simulink model "s_b4a4x32kf_26"  (R2018a)
settings: Solver=VariableStepDiscrete  StartTime=0.0  StopTime=10000  RelTol=1e-3
undefined symbols (not defined in the file): fft_stages, n_bits_ants, n_bits_xengs
libraries: xbsIndex_r4 x21247, casper_library_misc x37, casper_library_scopes x13, casper_library_delays x8, xbsReplacements_r4 x6, xps_library x4
(part 44 of 268)

== system s_b4a4x32kf_26/sys2/xeng_tvg ==
  sync : Inport
  data_in : Inport  Port=2
  valid_in : Inport  Port=3
  mcnti : Inport  Port=4
  Concat1 : xbsIndex_r4/Concat  num_inputs=4  dbl_ovrd=off  block_type=concat
      settings: SourceProductName=The database /home/jmanley/.matlab/R2018a/slblocks_master.db is locked, or a table in the database is locked. (database is locked)  block_version=10.1.3
  Constant1 : xbsIndex_r4/Constant  const=0.75  gui_display_data_type=Fixed-point  arith_type=Signed (2's comp)  n_bits=n_bits  bin_pt=n_bits-1  preci_type=Single  exp_width=8  frac_width=24  explicit_period=on  period=1  equ=P=C  opselect=C  inp2=PCIN>>17  opr=+  inp1=P  carry=CIN  dbl_ovrd=off  block_type=constant
      settings: SourceProductName=The database /home/jmanley/.matlab/R2018a/slblocks_master.db is locked, or a table in the database is locked. (database is locked)
  Constant13 : xbsIndex_r4/Constant  const=1  gui_display_data_type=Fixed-point  arith_type=Boolean  n_bits=1  bin_pt=0  preci_type=Single  exp_width=8  frac_width=24  explicit_period=on  period=1  equ=P=C  opselect=C  inp2=PCIN>>17  opr=+  inp1=P  carry=CIN  dbl_ovrd=off  block_type=constant
      settings: SourceProductName=The database /home/jmanley/.matlab/R2018a/slblocks_master.db is locked, or a table in the database is locked. (database is locked)
  Constant2 : xbsIndex_r4/Constant  const=0.125  gui_display_data_type=Fixed-point  arith_type=Signed (2's comp)  n_bits=n_bits  bin_pt=n_bits-1  preci_type=Single  exp_width=8  frac_width=24  explicit_period=on  period=1  equ=P=C  opselect=C  inp2=PCIN>>17  opr=+  inp1=P  carry=CIN  dbl_ovrd=off  block_type=constant
      settings: SourceProductName=The database /home/jmanley/.matlab/R2018a/slblocks_master.db is locked, or a table in the database is locked. (database is locked)
  Constant4 : xbsIndex_r4/Constant  const=-0.25  gui_display_data_type=Fixed-point  arith_type=Signed (2's comp)  n_bits=n_bits  bin_pt=n_bits-1  preci_type=Single  exp_width=8  frac_width=24  explicit_period=on  period=1  equ=P=C  opselect=C  inp2=PCIN>>17  opr=+  inp1=P  carry=CIN  dbl_ovrd=off  block_type=constant
      settings: SourceProductName=The database /home/jmanley/.matlab/R2018a/slblocks_master.db is locked, or a table in the database is locked. (database is locked)
  Constant7 : xbsIndex_r4/Constant  const=0.25  gui_display_data_type=Fixed-point  arith_type=Signed (2's comp)  n_bits=n_bits  bin_pt=n_bits-1  preci_type=Single  exp_width=8  frac_width=24  explicit_period=on  period=1  equ=P=C  opselect=C  inp2=PCIN>>17  opr=+  inp1=P  carry=CIN  dbl_ovrd=off  block_type=constant
      settings: SourceProductName=The database /home/jmanley/.matlab/R2018a/slblocks_master.db is locked, or a table in the database is locked. (database is locked)
  Counter : xbsIndex_r4/Counter  cnt_type=Free Running  cnt_to=Inf  operation=Up  start_count=0  cnt_by_val=1  arith_type=Unsigned  n_bits=x_int_bits + 1  bin_pt=0  load_pin=off  rst=on  en=off  explicit_period=off  period=1  use_behavioral_HDL=off  implementation=Fabric  use_rpm=on  dbl_ovrd=off  block_type=counter
      settings: SourceProductName=The database /home/jmanley/.matlab/R2018a/slblocks_master.db is locked, or a table in the database is locked. (database is locked)  xl_area=[0, 0, 0, 0, 0, 0, 0]
  Counter1 : xbsIndex_r4/Counter  cnt_type=Free Running  cnt_to=7  operation=Up  start_count=0  cnt_by_val=1  arith_type=Unsigned  n_bits=n_bits  bin_pt=0  load_pin=off  rst=on  en=on  explicit_period=off  period=1  use_behavioral_HDL=off  implementation=Fabric  use_rpm=on  dbl_ovrd=off  block_type=counter
      settings: SourceProductName=The database /home/jmanley/.matlab/R2018a/slblocks_master.db is locked, or a table in the database is locked. (database is locked)  xl_area=[0, 0, 0, 0, 0, 0, 0]
  Counter2 : xbsIndex_r4/Counter  cnt_type=Free Running  cnt_to=Inf  operation=Up  start_count=0  cnt_by_val=1  arith_type=Unsigned  n_bits=mcnt_period+1  bin_pt=0  load_pin=off  rst=on  en=on  explicit_period=off  period=1  use_behavioral_HDL=off  implementation=Fabric  use_rpm=on  dbl_ovrd=off  block_type=counter
      settings: SourceProductName=The database /home/jmanley/.matlab/R2018a/slblocks_master.db is locked, or a table in the database is locked. (database is locked)  xl_area=[0, 0, 0, 0, 0, 0, 0]
  Counter3 : xbsIndex_r4/Counter  cnt_type=Free Running  cnt_to=0  operation=Down  start_count=2^n_bits-1  cnt_by_val=1  arith_type=Unsigned  n_bits=n_bits  bin_pt=0  load_pin=off  rst=on  en=on  explicit_period=off  period=1  use_behavioral_HDL=off  implementation=Fabric  use_rpm=on  dbl_ovrd=off  block_type=counter
      settings: SourceProductName=The database /home/jmanley/.matlab/R2018a/slblocks_master.db is locked, or a table in the database is locked. (database is locked)  xl_area=[0, 0, 0, 0, 0, 0, 0]
  Counter4 : xbsIndex_r4/Counter  cnt_type=Free Running  cnt_to=Inf  operation=Up  start_count=2^sync_period - 2  cnt_by_val=1  arith_type=Unsigned  n_bits=sync_period+1  bin_pt=0  load_pin=off  rst=off  en=off  explicit_period=off  period=1  use_behavioral_HDL=off  implementation=Fabric  use_rpm=on  dbl_ovrd=off  block_type=counter
      settings: SourceProductName=The database /home/jmanley/.matlab/R2018a/slblocks_master.db is locked, or a table in the database is locked. (database is locked)  xl_area=[0, 0, 0, 0, 0, 0, 0]
  Counter5 : xbsIndex_r4/Counter  cnt_type=Free Running  cnt_to=Inf  operation=Up  start_count=0  cnt_by_val=mcnt_step  arith_type=Unsigned  n_bits=n_bits_mcnt  bin_pt=0  load_pin=off  rst=on  en=on  explicit_period=off  period=1  use_behavioral_HDL=off  implementation=Fabric  use_rpm=on  dbl_ovrd=off  block_type=counter
      settings: SourceProductName=The database /home/jmanley/.matlab/R2018a/slblocks_master.db is locked, or a table in the database is locked. (database is locked)  xl_area=[0, 0, 0, 0, 0, 0, 0]
  Counter6 : xbsIndex_r4/Counter  cnt_type=Free Running  cnt_to=Inf  operation=Up  start_count=0  cnt_by_val=1  arith_type=Unsigned  n_bits=x_int_bits + ant_bits + 1  bin_pt=0  load_pin=off  rst=on  en=off  explicit_period=off  period=1  use_behavioral_HDL=off  implementation=Fabric  use_rpm=on  dbl_ovrd=off  block_type=counter
      settings: SourceProductName=The database /home/jmanley/.matlab/R2018a/slblocks_master.db is locked, or a table in the database is locked. (database is locked)  xl_area=[0, 0, 0, 0, 0, 0, 0]
  Delay{1,3..18} (17 alike) : xbsIndex_r4/Delay  rst=off  infoeditControl=Selection of Reset will increase slice count due to use of real FFs and instead of SRLs  en=off  latency=1  reg_retiming=on  dbl_ovrd=off  block_type=delay
      settings: SourceProductName=The database /home/jmanley/.matlab/R2018a/slblocks_master.db is locked, or a table in the database is locked. (database is locked)  xl_area=[0, 0, 0, 0, 0, 0, 0]
  Delay2 : xbsIndex_r4/Delay  rst=off  infoeditControl=Selection of Reset will increase slice count due to use of real FFs and instead of SRLs  en=off  latency=2  reg_retiming=on  dbl_ovrd=off  block_type=delay
      settings: SourceProductName=The database /home/jmanley/.matlab/R2018a/slblocks_master.db is locked, or a table in the database is locked. (database is locked)  xl_area=[0, 0, 0, 0, 0, 0, 0]
  Mux1 : xbsIndex_r4/Mux  inputs=2  en=off  latency=0  precision=Full  arith_type="Signed  (2's comp)"  n_bits=8  bin_pt=2  quantization=Truncate  overflow=Wrap  dbl_ovrd=off  block_type=mux
      settings: SourceProductName=The database /home/jmanley/.matlab/R2018a/slblocks_master.db is locked, or a table in the database is locked. (database is locked)  xl_area=[0, 0, 0, 0, 0, 0, 0]
  Mux2 : xbsIndex_r4/Mux  inputs=2  en=off  latency=1  precision=Full  arith_type="Signed  (2's comp)"  n_bits=8  bin_pt=2  quantization=Truncate  overflow=Wrap  dbl_ovrd=off  block_type=mux
      settings: SourceProductName=The database /home/jmanley/.matlab/R2018a/slblocks_master.db is locked, or a table in the database is locked. (database is locked)  xl_area=[0, 0, 0, 0, 0, 0, 0]
  Mux3 : xbsIndex_r4/Mux  inputs=4  en=off  latency=1  precision=Full  arith_type="Signed  (2's comp)"  n_bits=8  bin_pt=2  quantization=Truncate  overflow=Wrap  dbl_ovrd=off  block_type=mux
      settings: SourceProductName=The database /home/jmanley/.matlab/R2018a/slblocks_master.db is locked, or a table in the database is locked. (database is locked)  xl_area=[0, 0, 0, 0, 0, 0, 0]
  Mux4 : xbsIndex_r4/Mux  inputs=2  en=off  latency=0  precision=Full  arith_type="Signed  (2's comp)"  n_bits=8  bin_pt=2  quantization=Truncate  overflow=Wrap  dbl_ovrd=off  block_type=mux
      settings: SourceProductName=The database /home/jmanley/.matlab/R2018a/slblocks_master.db is locked, or a table in the database is locked. (database is locked)  xl_area=[0, 0, 0, 0, 0, 0, 0]
  Slice1 : xbsIndex_r4/Slice  nbits=1  boolean_output=on  mode=Upper Bit Location + Width  bit1=0  base1=MSB of Input  bit0=x_int_bits  base0=LSB of Input  dbl_ovrd=off  block_type=slice
      settings: SourceProductName=The database /home/jmanley/.matlab/R2018a/slblocks_master.db is locked, or a table in the database is locked. (database is locked)  block_version=10.1.3
  Slice2 : xbsIndex_r4/Slice  nbits=1  boolean_output=on  mode=Lower Bit Location + Width  bit1=0  base1=MSB of Input  bit0=x_int_bits  base0=LSB of Input  dbl_ovrd=off  block_type=slice
      settings: SourceProductName=The database /home/jmanley/.matlab/R2018a/slblocks_master.db is locked, or a table in the database is locked. (database is locked)  infoedit="Extracts a given range of bits from each input sample and presents it at the output.  The output type is ordinarily unsigned with binary point at zero, but can be Boolean when the slice is one bit wide.<P><P>Hardware notes: In hardware this block costs nothing."  block_version=10.1.3
  Slice3 : xbsIndex_r4/Slice  nbits=2  boolean_output=off  mode=Lower Bit Location + Width  bit1=0  base1=MSB of Input  bit0=0  base0=LSB of Input  dbl_ovrd=off  block_type=slice
      settings: SourceProductName=The database /home/jmanley/.matlab/R2018a/slblocks_master.db is locked, or a table in the database is locked. (database is locked)  block_version=10.1.3
  Slice4 : xbsIndex_r4/Slice  nbits=1  boolean_output=on  mode=Lower Bit Location + Width  bit1=0  base1=MSB of Input  bit0=sync_period  base0=LSB of Input  dbl_ovrd=off  block_type=slice
      settings: SourceProductName=The database /home/jmanley/.matlab/R2018a/slblocks_master.db is locked, or a table in the database is locked. (database is locked)  infoedit="Extracts a given range of bits from each input sample and presents it at the output.  The output type is ordinarily unsigned with binary point at zero, but can be Boolean when the slice is one bit wide.<P><P>Hardware notes: In hardware this block costs nothing."  block_version=10.1.3
  Slice5 : xbsIndex_r4/Slice  nbits=1  boolean_output=on  mode=Upper Bit Location + Width  bit1=0  base1=MSB of Input  bit0=0  base0=LSB of Input  dbl_ovrd=off  block_type=slice
      settings: SourceProductName=The database /home/jmanley/.matlab/R2018a/slblocks_master.db is locked, or a table in the database is locked. (database is locked)  block_version=10.1.3
  ant_edge : Subsystem  mask(edge_detect){edge=Both, polarity=Active High, x_in=[0 0.08 0.08 0.16 0.16 0.24 0.24 0.32 0.32 0.4], y_in=[-1 -1  1  1  1  1  1  1  1  1], x_out=[0.6 0.68 0.68 0.76 0.76 0.84 0.84 0.92 0.92 1], y_out=[-1 -1  1  1 -1 -1 -1 -1 -1 -1]}
      mask prompts: edge "Edge Type"; polarity "Output Polarity"; x_in "Input X Positions"; y_in "Input Y Positions"; x_out "Output X Positions"; y_out "Output Y Positions"
      mask help: Output is active for one-cycle after each edge of the specified type (i.e. rising, falling or both).
      mask init: same as s_b4a4x32kf_26/edge_detect
      settings: AttributesFormatString=|
      | both edges
      | active high
      mask Help: Output is active for one-cycle after each edge of the specified type (i.e. rising, falling, or both).  Latency is zero.
      mask TypeOptions edge: Rising | Falling | Both
      mask TypeOptions polarity: Active High | Active Low
      mask Display:
      | plot(x_in_num,0.5+y_in_num*0.2);
      | plot(x_out_num,0.5+y_out_num*0.2);
  block_edge : Subsystem  mask(edge_detect){edge=Both, polarity=Active High, x_in=[0 0.08 0.08 0.16 0.16 0.24 0.24 0.32 0.32 0.4], y_in=[-1 -1  1  1  1  1  1  1  1  1], x_out=[0.6 0.68 0.68 0.76 0.76 0.84 0.84 0.92 0.92 1], y_out=[-1 -1  1  1 -1 -1 -1 -1 -1 -1]}
      mask prompts: edge "Edge Type"; polarity "Output Polarity"; x_in "Input X Positions"; y_in "Input Y Positions"; x_out "Output X Positions"; y_out "Output Y Positions"
      mask help: Output is active for one-cycle after each edge of the specified type (i.e. rising, falling or both).
      mask init: same as s_b4a4x32kf_26/edge_detect
      settings: AttributesFormatString=|
      | both edges
      | active high
      mask Help: Output is active for one-cycle after each edge of the specified type (i.e. rising, falling, or both).  Latency is zero.
      mask TypeOptions edge: Rising | Falling | Both
      mask TypeOptions polarity: Active High | Active Low
      mask Display:
      | plot(x_in_num,0.5+y_in_num*0.2);
      | plot(x_out_num,0.5+y_out_num*0.2);
  bus_create : Subsystem  mask(bus_create){inputNum=4}
      mask prompts: inputNum "Number of inputs:"
      mask init:
      | bus_create_init(gcb,...
      |     'inputNum', inputNum);
  cont : Subsystem  Tag=xps:sw_reg  AncestorBlock=xps_library/Memory/software_register  mask(swreg){io_dir=From Processor, io_delay=0, init_val=0, sample_period=1, names=reg, bitwidths=32, bin_pts=0, arith_types=0, sim_port=off, show_format=on}
      mask prompts: io_dir "I/O direction"; io_delay "I/O delay"; init_val "Initial Value"; sample_period "Sample period"; names "Bitfield names [msb...lsb]"; bitwidths "Bitfield widths"; bin_pts "Bitfield binary pts"; arith_types "Bitfield types, ufix=0, fix=1, bool=2"; sim_port "Provide sim input/output?"; show_format "Print format string?"
      mask help: A 32-bit software-accessible register. Can be divided into bitfields of varying widths and types using the fields in the block mask.
      mask init:
      | swreg_init(gcb)
      settings: AttributesFormatString=1input:uf32.0 = 32 bits
      mask TypeOptions io_dir: To Processor | From Processor
      mask Callback io_dir:
      | mask_enables = get_param(gcb, 'MaskEnables');
      | mask_names = get_param(gcb, 'MaskNames');
      | if strcmp(get_param(gcb, 'io_dir'), 'To Processor'),
      |     mask_enables{ismember(mask_names, 'sample_period')} = 'off';
      | else
      |     mask_enables{ismember(mask_names, 'sample_period')} = 'on';
      | end
      | set_param(gcb, 'MaskEnables', mask_enables);
      mask DialogControl ParameterTabVar0 Prompt: Setup
  edge1 : Subsystem  mask(edge_detect){edge=Both, polarity=Active High, x_in=[0 0.08 0.08 0.16 0.16 0.24 0.24 0.32 0.32 0.4], y_in=[-1 -1  1  1  1  1  1  1  1  1], x_out=[0.6 0.68 0.68 0.76 0.76 0.84 0.84 0.92 0.92 1], y_out=[-1 -1  1  1 -1 -1 -1 -1 -1 -1]}
      mask prompts: edge "Edge Type"; polarity "Output Polarity"; x_in "Input X Positions"; y_in "Input Y Positions"; x_out "Output X Positions"; y_out "Output Y Positions"
      mask help: Output is active for one-cycle after each edge of the specified type (i.e. rising, falling or both).
      mask init: same as s_b4a4x32kf_26/edge_detect
      settings: AttributesFormatString=|
      | both edges
      | active high
      mask Help: Output is active for one-cycle after each edge of the specified type (i.e. rising, falling, or both).  Latency is zero.
      mask TypeOptions edge: Rising | Falling | Both
      mask TypeOptions polarity: Active High | Active Low
      mask Display:
      | plot(x_in_num,0.5+y_in_num*0.2);
      | plot(x_out_num,0.5+y_out_num*0.2);
  ins_vect_loc0 : Subsystem  Tag=xps:sw_reg  AncestorBlock=xps_library/Memory/software_register  mask(swreg){io_dir=From Processor, io_delay=0, init_val=0, sample_period=1, names=reg, bitwidths=32, bin_pts=0, arith_types=0, sim_port=on, show_format=on}
      mask prompts: io_dir "I/O direction"; io_delay "I/O delay"; init_val "Initial Value"; sample_period "Sample period"; names "Bitfield names [msb...lsb]"; bitwidths "Bitfield widths"; bin_pts "Bitfield binary pts"; arith_types "Bitfield types, ufix=0, fix=1, bool=2"; sim_port "Provide sim input/output?"; show_format "Print format string?"
      mask help: A 32-bit software-accessible register. Can be divided into bitfields of varying widths and types using the fields in the block mask.
      mask init:
      | swreg_init(gcb)
      settings: AttributesFormatString=1input:uf32.0 = 32 bits
      mask TypeOptions io_dir: To Processor | From Processor
      mask Callback io_dir:
      | mask_enables = get_param(gcb, 'MaskEnables');
      | mask_names = get_param(gcb, 'MaskNames');
      | if strcmp(get_param(gcb, 'io_dir'), 'To Processor'),
      |     mask_enables{ismember(mask_names, 'sample_period')} = 'off';
      | else
      |     mask_enables{ismember(mask_names, 'sample_period')} = 'on';
      | end
      | set_param(gcb, 'MaskEnables', mask_enables);
      mask DialogControl ParameterTabVar0 Prompt: Setup
  ins_vect_loc1 : Subsystem  Tag=xps:sw_reg  AncestorBlock=xps_library/Memory/software_register  mask(swreg){io_dir=From Processor, io_delay=0, init_val=0, sample_period=1, names=reg, bitwidths=32, bin_pts=0, arith_types=0, sim_port=on, show_format=on}
      mask prompts: io_dir "I/O direction"; io_delay "I/O delay"; init_val "Initial Value"; sample_period "Sample period"; names "Bitfield names [msb...lsb]"; bitwidths "Bitfield widths"; bin_pts "Bitfield binary pts"; arith_types "Bitfield types, ufix=0, fix=1, bool=2"; sim_port "Provide sim input/output?"; show_format "Print format string?"
      mask help: A 32-bit software-accessible register. Can be divided into bitfields of varying widths and types using the fields in the block mask.
      mask init:
      | swreg_init(gcb)
      settings: AttributesFormatString=1input:uf32.0 = 32 bits
      mask TypeOptions io_dir: To Processor | From Processor
      mask Callback io_dir:
      | mask_enables = get_param(gcb, 'MaskEnables');
      | mask_names = get_param(gcb, 'MaskNames');
      | if strcmp(get_param(gcb, 'io_dir'), 'To Processor'),
      |     mask_enables{ismember(mask_names, 'sample_period')} = 'off';
      | else
      |     mask_enables{ismember(mask_names, 'sample_period')} = 'on';
      | end
      | set_param(gcb, 'MaskEnables', mask_enables);
      mask DialogControl ParameterTabVar0 Prompt: Setup
  ins_vect_val0 : Subsystem  Tag=xps:sw_reg  AncestorBlock=xps_library/Memory/software_register  mask(swreg){io_dir=From Processor, io_delay=0, init_val=0, sample_period=1, names=reg, bitwidths=32, bin_pts=0, arith_types=0, sim_port=on, show_format=on}
      mask prompts: io_dir "I/O direction"; io_delay "I/O delay"; init_val "Initial Value"; sample_period "Sample period"; names "Bitfield names [msb...lsb]"; bitwidths "Bitfield widths"; bin_pts "Bitfield binary pts"; arith_types "Bitfield types, ufix=0, fix=1, bool=2"; sim_port "Provide sim input/output?"; show_format "Print format string?"
      mask help: A 32-bit software-accessible register. Can be divided into bitfields of varying widths and types using the fields in the block mask.
      mask init:
      | swreg_init(gcb)
      settings: AttributesFormatString=1input:uf32.0 = 32 bits
      mask TypeOptions io_dir: To Processor | From Processor
      mask Callback io_dir:
      | mask_enables = get_param(gcb, 'MaskEnables');
      | mask_names = get_param(gcb, 'MaskNames');
      | if strcmp(get_param(gcb, 'io_dir'), 'To Processor'),
      |     mask_enables{ismember(mask_names, 'sample_period')} = 'off';
      | else
      |     mask_enables{ismember(mask_names, 'sample_period')} = 'on';
      | end
      | set_param(gcb, 'MaskEnables', mask_enables);
      mask DialogControl ParameterTabVar0 Prompt: Setup
  ins_vect_val1 : Subsystem  Tag=xps:sw_reg  AncestorBlock=xps_library/Memory/software_register  mask(swreg){io_dir=From Processor, io_delay=0, init_val=0, sample_period=1, names=reg, bitwidths=32, bin_pts=0, arith_types=0, sim_port=on, show_format=on}
      mask prompts: io_dir "I/O direction"; io_delay "I/O delay"; init_val "Initial Value"; sample_period "Sample period"; names "Bitfield names [msb...lsb]"; bitwidths "Bitfield widths"; bin_pts "Bitfield binary pts"; arith_types "Bitfield types, ufix=0, fix=1, bool=2"; sim_port "Provide sim input/output?"; show_format "Print format string?"
      mask help: A 32-bit software-accessible register. Can be divided into bitfields of varying widths and types using the fields in the block mask.
      mask init:
      | swreg_init(gcb)
      settings: AttributesFormatString=1input:uf32.0 = 32 bits
      mask TypeOptions io_dir: To Processor | From Processor
      mask Callback io_dir:
      | mask_enables = get_param(gcb, 'MaskEnables');
      | mask_names = get_param(gcb, 'MaskNames');
      | if strcmp(get_param(gcb, 'io_dir'), 'To Processor'),
      |     mask_enables{ismember(mask_names, 'sample_period')} = 'off';
      | else
      |     mask_enables{ismember(mask_names, 'sample_period')} = 'on';
      | end
      | set_param(gcb, 'MaskEnables', mask_enables);
      mask DialogControl ParameterTabVar0 Prompt: Setup
  ins_vector0 : Subsystem  mask{num_vectors=2^(x_int_bits + ant_bits)}
      mask prompts: num_vectors "number of vectors"
      mask init:
      | fmtstr = sprintf('Vector Length: %d', num_vectors);
      | set_param(gcb, 'AttributesFormatString', fmtstr);
      settings: AttributesFormatString=Vector Length: 1024
  ins_vector1 : Subsystem  mask{num_vectors=2^(x_int_bits + ant_bits)}
      mask prompts: num_vectors "number of vectors"
      mask init:
      | fmtstr = sprintf('Vector Length: %d', num_vectors);
      | set_param(gcb, 'AttributesFormatString', fmtstr);
      settings: AttributesFormatString=Vector Length: 1024
  master_reset_sim1 : Constant  Value=1000
  master_reset_sim10 : Constant  Value=1000
  master_reset_sim11 : Constant  Value=127
  master_reset_sim2 : Constant  Value=127
  tvg_edge : Subsystem  mask(edge_detect){edge=Rising, polarity=Active High, x_in=[0 0.08 0.08 0.16 0.16 0.24 0.24 0.32 0.32 0.4], y_in=[-1 -1  1  1  1  1  1  1  1  1], x_out=[0.6 0.68 0.68 0.76 0.76 0.84 0.84 0.92 0.92 1], y_out=[-1 -1  1  1 -1 -1 -1 -1 -1 -1]}
      mask prompts: edge "Edge Type"; polarity "Output Polarity"; x_in "Input X Positions"; y_in "Input Y Positions"; x_out "Output X Positions"; y_out "Output Y Positions"
      mask help: Output is active for one-cycle after each edge of the specified type (i.e. rising, falling or both).
      mask init: same as s_b4a4x32kf_26/edge_detect
      settings: AttributesFormatString=|
      | rising edges
      | active high
      mask Help: Output is active for one-cycle after each edge of the specified type (i.e. rising, falling, or both).  Latency is zero.
      mask TypeOptions edge: Rising | Falling | Both
      mask TypeOptions polarity: Active High | Active Low
      mask Display:
      | plot(x_in_num,0.5+y_in_num*0.2);
      | plot(x_out_num,0.5+y_out_num*0.2);
  window_edge : Subsystem  mask(edge_detect){edge=Both, polarity=Active High, x_in=[0 0.08 0.08 0.16 0.16 0.24 0.24 0.32 0.32 0.4], y_in=[-1 -1  1  1  1  1  1  1  1  1], x_out=[0.6 0.68 0.68 0.76 0.76 0.84 0.84 0.92 0.92 1], y_out=[-1 -1  1  1 -1 -1 -1 -1 -1 -1]}
      mask prompts: edge "Edge Type"; polarity "Output Polarity"; x_in "Input X Positions"; y_in "Input Y Positions"; x_out "Output X Positions"; y_out "Output Y Positions"
      mask help: Output is active for one-cycle after each edge of the specified type (i.e. rising, falling or both).
      mask init: same as s_b4a4x32kf_26/edge_detect
      settings: AttributesFormatString=|
      | both edges
      | active high
      mask Help: Output is active for one-cycle after each edge of the specified type (i.e. rising, falling, or both).  Latency is zero.
      mask TypeOptions edge: Rising | Falling | Both
      mask TypeOptions polarity: Active High | Active Low
      mask Display:
      | plot(x_in_num,0.5+y_in_num*0.2);
      | plot(x_out_num,0.5+y_out_num*0.2);
  sync_out : Outport
  data_out : Outport  Port=2
  valid_out : Outport  Port=3
  mcnto : Outport  Port=4
  wires:
  Constant2/1 -> bus_create/4(in4)
  Constant1/1 -> bus_create/2(in2)
  Constant7/1 -> bus_create/1(in1)
  Constant4/1 -> bus_create/3(in3)
  Counter1/1 -> Concat1/1, Concat1/3
  Slice2/1 -> ant_edge/1(in)
  Counter/1 -> Slice2/1
  Concat1/1 -> Delay4/1
  data_in/1 -> Delay2/1
  Delay2/1 -> Mux3/2
  [xeng_tvg_data_sel] -> Slice3/1
  Delay6/1 -> Mux3/1
  bus_create/1(bus_out) -> Mux3/4
  Counter3/1 -> Concat1/2, Concat1/4
  Delay1/1 -> Delay7/1
  Delay8/1 -> Delay1/1
  Delay4/1 -> Mux3/3
  [xeng_tvg_val_sel] -> Mux4/1
  Slice4/1 -> edge1/1(in)
  Counter4/1 -> Slice4/1
  sync/1 -> Mux4/2
  Mux4/1 -> Delay8/1
  edge1/1(out) -> Mux4/3
  valid_in/1 -> Mux1/2
  Mux1/1 -> Counter/1, Counter6/1, Delay9/1
  [xeng_tvg_val_sel] -> Mux1/1
  Delay9/1 -> Counter2/2, Delay3/1
  mcnti/1 -> Delay14/1
  Constant13/1 -> Mux1/3
  Delay15/1 -> Mux2/2
  Delay3/1 -> Delay5/1
  Delay14/1 -> Delay15/1
  tvg_edge/1(out) -> Counter5/1, Counter2/1
  [xeng_tvg_mcnt_sel] -> Mux2/1
  [xeng_tvg_mcnt_sel] -> tvg_edge/1(in)
  Counter2/1 -> Slice1/1
  Counter5/1 -> Mux2/3
  Slice1/1 -> Delay11/1
  block_edge/1(out) -> Counter5/2
  Delay11/1 -> block_edge/1(in)
  master_reset_sim11/1 -> ins_vect_loc0/1(sim_1)
  ins_vect_loc0/1(in_reg) -> Delay16/1
  master_reset_sim10/1 -> ins_vect_val0/1(sim_1)
  ins_vect_val0/1(in_reg) -> Delay13/1
  Mux2/1 -> ins_vector0/7(mcnt_in)
  Delay7/1 -> ins_vector0/1(sync_in)
  Mux3/1 -> ins_vector0/2(data_in)
  Delay5/1 -> ins_vector0/3(valid_in)
  master_reset_sim2/1 -> ins_vect_loc1/1(sim_1)
  ins_vect_loc1/1(in_reg) -> Delay17/1
  master_reset_sim1/1 -> ins_vect_val1/1(sim_1)
  ins_vect_val1/1(in_reg) -> Delay18/1
  ins_vector0/1(sync_out) -> ins_vector1/1(sync_in)
  ins_vector0/2(data) -> ins_vector1/2(data_in)
  ins_vector0/3(valid_out) -> ins_vector1/3(valid_in)
  ins_vector0/4(mcnt_out) -> ins_vector1/7(mcnt_in)
  ins_vector1/3(valid_out) -> valid_out/1
  ins_vector1/2(data) -> data_out/1
  ins_vector1/4(mcnt_out) -> mcnto/1
  ins_vector1/1(sync_out) -> sync_out/1
  Slice3/1 -> Delay6/1
  cont/1(in_reg) -> Delay12/1
  Delay10/1 -> Mux3/5
  Delay12/1 -> Delay10/1
  Delay13/1 -> ins_vector0/5(value)
  Delay16/1 -> ins_vector0/4(vector)
  Delay17/1 -> ins_vector1/4(vector)
  Delay18/1 -> ins_vector1/5(value)
  [xengtvg_inj_vector] -> ins_vector0/6(enable)
  [xengtvg_inj_vector] -> ins_vector1/6(enable)
  Slice5/1 -> window_edge/1(in)
  Counter6/1 -> Slice5/1
  ant_edge/1(out) -> Counter1/2, Counter3/2
  window_edge/1(out) -> Counter3/1, Counter1/1

== system s_b4a4x32kf_26/sys3/31->32 ==
  din : Inport
  bussify : Subsystem  AncestorBlock=casper_library_flow_control/bus_create  mask(bus_create){inputNum=8}
      mask prompts: inputNum "Number of inputs:"
      mask init:
      | bus_create_init(gcb,...
      |     'inputNum', inputNum);
  conv1 : Subsystem  AncestorBlock=casper_library_misc/convert  mask(convert){bin_pt_in=0, n_bits_out=32, bin_pt_out=0, quantization=Truncate, overflow=Wrap, csp_latency=0}
      mask prompts: bin_pt_in "Binary Point In"; n_bits_out "Bit Width Out"; bin_pt_out "Binary Point Out"; csp_latency "Latency"
      mask help:
      | Convert input value to the specified bit width and precision.
      |
      | Does not support upscaling number of fractional bits (eg 8_5 to 8_4 is ok, but not 8_4 to 8_5).
      mask init: same as s_b4a4x32kf_26/sys0/31->32/conv1
      settings: AttributesFormatString=|
      | N_0 ==> 32_0
      | truncate, wrap
      | latency = 0
      mask Help:
      | <pre>
      | Description::
      | 
      | Outputs converted version of the input.
      | 
      | Mask Parameters::
      | 
      | Binary Point In (bin_pt_in): Specifies the binary point location in the input.
      | 
      | Bit Width Out (n_bits_out): Specifies the width of the output.
      | 
      | Binary Point Out (bin_pt_out): Specifies the binary point location in the output.
      | 
      | Quantization (quantization): Specifies quantization handling.
      | 
      | Overflow (overflow): Specifies overflow handling.
      | 
      | Latency (latency): Specifies the latency of the underlying adder block, which is the overall
      | latency of this block as well.
      | </pre>
      mask TypeOptions quantization: Truncate | Round  (unbiased: +/- Inf) | Round  (unbiased: Even Values) | Round  (unbiased: Zero) | Round  (unbiased: Odd Values) | Round  (biased: Up) | Round  (biased: Down)
      mask TypeOptions overflow: Wrap | Saturate | Error
  conv2 : Subsystem  AncestorBlock=casper_library_misc/convert  mask(convert){bin_pt_in=0, n_bits_out=32, bin_pt_out=0, quantization=Truncate, overflow=Wrap, csp_latency=0}
      mask prompts: bin_pt_in "Binary Point In"; n_bits_out "Bit Width Out"; bin_pt_out "Binary Point Out"; csp_latency "Latency"
      mask help:
      | Convert input value to the specified bit width and precision.
      |
      | Does not support upscaling number of fractional bits (eg 8_5 to 8_4 is ok, but not 8_4 to 8_5).
      mask init: same as s_b4a4x32kf_26/sys0/31->32/conv1
      settings: AttributesFormatString=|
      | N_0 ==> 32_0
      | truncate, wrap
      | latency = 0
      mask Help:
      | <pre>
      | Description::
      | 
      | Outputs converted version of the input.
      | 
      | Mask Parameters::
      | 
      | Binary Point In (bin_pt_in): Specifies the binary point location in the input.
      | 
      | Bit Width Out (n_bits_out): Specifies the width of the output.
      | 
      | Binary Point Out (bin_pt_out): Specifies the binary point location in the output.
      | 
      | Quantization (quantization): Specifies quantization handling.
      | 
      | Overflow (overflow): Specifies overflow handling.
      | 
      | Latency (latency): Specifies the latency of the underlying adder block, which is the overall
      | latency of this block as well.
      | </pre>
      mask TypeOptions quantization: Truncate | Round  (unbiased: +/- Inf) | Round  (unbiased: Even Values) | Round  (unbiased: Zero) | Round  (unbiased: Odd Values) | Round  (biased: Up) | Round  (biased: Down)
      mask TypeOptions overflow: Wrap | Saturate | Error
  conv3 : Subsystem  AncestorBlock=casper_library_misc/convert  mask(convert){bin_pt_in=0, n_bits_out=32, bin_pt_out=0, quantization=Truncate, overflow=Wrap, csp_latency=0}
      mask prompts: bin_pt_in "Binary Point In"; n_bits_out "Bit Width Out"; bin_pt_out "Binary Point Out"; csp_latency "Latency"
      mask help:
      | Convert input value to the specified bit width and precision.
      |
      | Does not support upscaling number of fractional bits (eg 8_5 to 8_4 is ok, but not 8_4 to 8_5).
      mask init: same as s_b4a4x32kf_26/sys0/31->32/conv1
      settings: AttributesFormatString=|
      | N_0 ==> 32_0
      | truncate, wrap
      | latency = 0
      mask Help:
      | <pre>
      | Description::
      | 
      | Outputs converted version of the input.
      | 
      | Mask Parameters::
      | 
      | Binary Point In (bin_pt_in): Specifies the binary point location in the input.
      | 
      | Bit Width Out (n_bits_out): Specifies the width of the output.
      | 
      | Binary Point Out (bin_pt_out): Specifies the binary point location in the output.
      | 
      | Quantization (quantization): Specifies quantization handling.
      | 
      | Overflow (overflow): Specifies overflow handling.
      | 
      | Latency (latency): Specifies the latency of the underlying adder block, which is the overall
      | latency of this block as well.
      | </pre>
      mask TypeOptions quantization: Truncate | Round  (unbiased: +/- Inf) | Round  (unbiased: Even Values) | Round  (unbiased: Zero) | Round  (unbiased: Odd Values) | Round  (biased: Up) | Round  (biased: Down)
      mask TypeOptions overflow: Wrap | Saturate | Error
  conv4 : Subsystem  AncestorBlock=casper_library_misc/convert  mask(convert){bin_pt_in=0, n_bits_out=32, bin_pt_out=0, quantization=Truncate, overflow=Wrap, csp_latency=0}
      mask prompts: bin_pt_in "Binary Point In"; n_bits_out "Bit Width Out"; bin_pt_out "Binary Point Out"; csp_latency "Latency"
      mask help:
      | Convert input value to the specified bit width and precision.
      |
      | Does not support upscaling number of fractional bits (eg 8_5 to 8_4 is ok, but not 8_4 to 8_5).
      mask init: same as s_b4a4x32kf_26/sys0/31->32/conv1
      settings: AttributesFormatString=|
      | N_0 ==> 32_0
      | truncate, wrap
      | latency = 0
      mask Help:
      | <pre>
      | Description::
      | 
      | Outputs converted version of the input.
      | 
      | Mask Parameters::
      | 
      | Binary Point In (bin_pt_in): Specifies the binary point location in the input.
      | 
      | Bit Width Out (n_bits_out): Specifies the width of the output.
      | 
      | Binary Point Out (bin_pt_out): Specifies the binary point location in the output.
      | 
      | Quantization (quantization): Specifies quantization handling.
      | 
      | Overflow (overflow): Specifies overflow handling.
      | 
      | Latency (latency): Specifies the latency of the underlying adder block, which is the overall
      | latency of this block as well.
      | </pre>
      mask TypeOptions quantization: Truncate | Round  (unbiased: +/- Inf) | Round  (unbiased: Even Values) | Round  (unbiased: Zero) | Round  (unbiased: Odd Values) | Round  (biased: Up) | Round  (biased: Down)
      mask TypeOptions overflow: Wrap | Saturate | Error
  conv5 : Subsystem  AncestorBlock=casper_library_misc/convert  mask(convert){bin_pt_in=0, n_bits_out=32, bin_pt_out=0, quantization=Truncate, overflow=Wrap, csp_latency=0}
      mask prompts: bin_pt_in "Binary Point In"; n_bits_out "Bit Width Out"; bin_pt_out "Binary Point Out"; csp_latency "Latency"
      mask help:
      | Convert input value to the specified bit width and precision.
      |
      | Does not support upscaling number of fractional bits (eg 8_5 to 8_4 is ok, but not 8_4 to 8_5).
      mask init: same as s_b4a4x32kf_26/sys0/31->32/conv1
      settings: AttributesFormatString=|
      | N_0 ==> 32_0
      | truncate, wrap
      | latency = 0
      mask Help:
      | <pre>
      | Description::
      | 
      | Outputs converted version of the input.
      | 
      | Mask Parameters::
      | 
      | Binary Point In (bin_pt_in): Specifies the binary point location in the input.
      | 
      | Bit Width Out (n_bits_out): Specifies the width of the output.
      | 
      | Binary Point Out (bin_pt_out): Specifies the binary point location in the output.
      | 
      | Quantization (quantization): Specifies quantization handling.
      | 
      | Overflow (overflow): Specifies overflow handling.
      | 
      | Latency (latency): Specifies the latency of the underlying adder block, which is the overall
      | latency of this block as well.
      | </pre>
      mask TypeOptions quantization: Truncate | Round  (unbiased: +/- Inf) | Round  (unbiased: Even Values) | Round  (unbiased: Zero) | Round  (unbiased: Odd Values) | Round  (biased: Up) | Round  (biased: Down)
      mask TypeOptions overflow: Wrap | Saturate | Error
  conv6 : Subsystem  AncestorBlock=casper_library_misc/convert  mask(convert){bin_pt_in=0, n_bits_out=32, bin_pt_out=0, quantization=Truncate, overflow=Wrap, csp_latency=0}
      mask prompts: bin_pt_in "Binary Point In"; n_bits_out "Bit Width Out"; bin_pt_out "Binary Point Out"; csp_latency "Latency"
      mask help:
      | Convert input value to the specified bit width and precision.
      |
      | Does not support upscaling number of fractional bits (eg 8_5 to 8_4 is ok, but not 8_4 to 8_5).
      mask init: same as s_b4a4x32kf_26/sys0/31->32/conv1
      settings: AttributesFormatString=|
      | N_0 ==> 32_0
      | truncate, wrap
      | latency = 0
      mask Help:
      | <pre>
      | Description::
      | 
      | Outputs converted version of the input.
      | 
      | Mask Parameters::
      | 
      | Binary Point In (bin_pt_in): Specifies the binary point location in the input.
      | 
      | Bit Width Out (n_bits_out): Specifies the width of the output.
      | 
      | Binary Point Out (bin_pt_out): Specifies the binary point location in the output.
      | 
      | Quantization (quantization): Specifies quantization handling.
      | 
      | Overflow (overflow): Specifies overflow handling.
      | 
      | Latency (latency): Specifies the latency of the underlying adder block, which is the overall
      | latency of this block as well.
      | </pre>
      mask TypeOptions quantization: Truncate | Round  (unbiased: +/- Inf) | Round  (unbiased: Even Values) | Round  (unbiased: Zero) | Round  (unbiased: Odd Values) | Round  (biased: Up) | Round  (biased: Down)
      mask TypeOptions overflow: Wrap | Saturate | Error
  conv7 : Subsystem  AncestorBlock=casper_library_misc/convert  mask(convert){bin_pt_in=0, n_bits_out=32, bin_pt_out=0, quantization=Truncate, overflow=Wrap, csp_latency=0}
      mask prompts: bin_pt_in "Binary Point In"; n_bits_out "Bit Width Out"; bin_pt_out "Binary Point Out"; csp_latency "Latency"
      mask help:
      | Convert input value to the specified bit width and precision.
      |
      | Does not support upscaling number of fractional bits (eg 8_5 to 8_4 is ok, but not 8_4 to 8_5).
      mask init: same as s_b4a4x32kf_26/sys0/31->32/conv1
      settings: AttributesFormatString=|
      | N_0 ==> 32_0
      | truncate, wrap
      | latency = 0
      mask Help:
      | <pre>
      | Description::
      | 
      | Outputs converted version of the input.
      | 
      | Mask Parameters::
      | 
      | Binary Point In (bin_pt_in): Specifies the binary point location in the input.
      | 
      | Bit Width Out (n_bits_out): Specifies the width of the output.
      | 
      | Binary Point Out (bin_pt_out): Specifies the binary point location in the output.
      | 
      | Quantization (quantization): Specifies quantization handling.
      | 
      | Overflow (overflow): Specifies overflow handling.
      | 
      | Latency (latency): Specifies the latency of the underlying adder block, which is the overall
      | latency of this block as well.
      | </pre>
      mask TypeOptions quantization: Truncate | Round  (unbiased: +/- Inf) | Round  (unbiased: Even Values) | Round  (unbiased: Zero) | Round  (unbiased: Odd Values) | Round  (biased: Up) | Round  (biased: Down)
      mask TypeOptions overflow: Wrap | Saturate | Error
  conv8 : Subsystem  AncestorBlock=casper_library_misc/convert  mask(convert){bin_pt_in=0, n_bits_out=32, bin_pt_out=0, quantization=Truncate, overflow=Wrap, csp_latency=0}
      mask prompts: bin_pt_in "Binary Point In"; n_bits_out "Bit Width Out"; bin_pt_out "Binary Point Out"; csp_latency "Latency"
      mask help:
      | Convert input value to the specified bit width and precision.
      |
      | Does not support upscaling number of fractional bits (eg 8_5 to 8_4 is ok, but not 8_4 to 8_5).
      mask init: same as s_b4a4x32kf_26/sys0/31->32/conv1
      settings: AttributesFormatString=|
      | N_0 ==> 32_0
      | truncate, wrap
      | latency = 0
      mask Help:
      | <pre>
      | Description::
      | 
      | Outputs converted version of the input.
      | 
      | Mask Parameters::
      | 
      | Binary Point In (bin_pt_in): Specifies the binary point location in the input.
      | 
      | Bit Width Out (n_bits_out): Specifies the width of the output.
      | 
      | Binary Point Out (bin_pt_out): Specifies the binary point location in the output.
      | 
      | Quantization (quantization): Specifies quantization handling.
      | 
      | Overflow (overflow): Specifies overflow handling.
      | 
      | Latency (latency): Specifies the latency of the underlying adder block, which is the overall
      | latency of this block as well.
      | </pre>
      mask TypeOptions quantization: Truncate | Round  (unbiased: +/- Inf) | Round  (unbiased: Even Values) | Round  (unbiased: Zero) | Round  (unbiased: Odd Values) | Round  (biased: Up) | Round  (biased: Down)
      mask TypeOptions overflow: Wrap | Saturate | Error
  debus : Subsystem  AncestorBlock=casper_library_flow_control/bus_expand  mask(bus_expand){mode=divisions of arbitrary size, outputNum=1, outputWidth=[31 31 31 31 31 31 31 31], outputBinaryPt=[0 0 0 0 0 0 0 0], outputArithmeticType=[1 1 1 1 1 1 1 1], show_format=on, outputToWorkspace=off, variablePrefix=, outputToModelAsWell=on}
      mask prompts: outputNum "Number of outputs:"; outputWidth "Output width [msb ... lsb]:"; outputBinaryPt "Output binary point position [msb ... lsb]:"; outputArithmeticType "Output arithmetic type (ufix=0, fix=1, bool=2) [msb ... lsb]:"; show_format "Print format string?"; outputToWorkspace "Output to workspace?"; variablePrefix "Variable name prefix:"; outputToModelAsWell "Output to model as well?"
      mask help:
      | Expands a 'bus' made using a bus_create or Xilinx
      | concat block.
      | The input will be divided into the specified number
      | of outputs with the specified arithmetic types.
      | Divisions are made from most significant bit.
      mask init: same as s_b4a4x32kf_26/bus_expand
      settings: AttributesFormatString=8 outputs: f31.0,f31.0,f31.0,f31.0,f31.0,f31.0,f31.0,f31.0,
      mask TypeOptions mode: divisions of equal size | divisions of arbitrary size
      mask Callback mode: bus_expand_callback();
      mask Callback outputWidth: bus_expand_callback();
      mask Callback outputToWorkspace: bus_expand_callback();
  dout : Outport
  wires:
  din/1 -> debus/1(bus_in)
  debus/1(msb_out8) -> conv1/1(in)
  debus/2(out7) -> conv2/1(in)
  debus/3(out6) -> conv3/1(in)
  debus/4(out5) -> conv4/1(in)
  debus/5(out4) -> conv5/1(in)
  debus/6(out3) -> conv6/1(in)
  debus/7(out2) -> conv7/1(in)
  debus/8(lsb_out1) -> conv8/1(in)
  conv1/1(out) -> bussify/1(in1)
  conv2/1(out) -> bussify/2(in2)
  conv3/1(out) -> bussify/3(in3)
  conv4/1(out) -> bussify/4(in4)
  conv5/1(out) -> bussify/5(in5)
  conv6/1(out) -> bussify/6(in6)
  conv7/1(out) -> bussify/7(in7)
  conv8/1(out) -> bussify/8(in8)
  bussify/1(bus_out) -> dout/1

== system s_b4a4x32kf_26/sys3/Delay10 ==
  d : Inport
  Register0 : xbsIndex_r4/Register  init=0  rst=off  en=off  dbl_ovrd=off  block_type=register
      settings: SourceProductName=The database /home/jmanley/.matlab/R2018a/slblocks_master.db is locked, or a table in the database is locked. (database is locked)  block_version=11.4
  Register1 : xbsIndex_r4/Register  init=0  rst=off  en=off  dbl_ovrd=off  block_type=register
      settings: SourceProductName=The database /home/jmanley/.matlab/R2018a/slblocks_master.db is locked, or a table in the database is locked. (database is locked)  block_version=11.4
  q : Outport
  wires:
  Register0/1 -> Register1/1
  d/1 -> Register0/1
  Register1/1 -> q/1

== system s_b4a4x32kf_26/sys3/Delay11 ==
  d : Inport
  Register0 : xbsIndex_r4/Register  init=0  rst=off  en=off  dbl_ovrd=off  block_type=register
      settings: SourceProductName=The database /home/jmanley/.matlab/R2018a/slblocks_master.db is locked, or a table in the database is locked. (database is locked)  block_version=11.4
  Register1 : xbsIndex_r4/Register  init=0  rst=off  en=off  dbl_ovrd=off  block_type=register
      settings: SourceProductName=The database /home/jmanley/.matlab/R2018a/slblocks_master.db is locked, or a table in the database is locked. (database is locked)  block_version=11.4
  q : Outport
  wires:
  Register0/1 -> Register1/1
  d/1 -> Register0/1
  Register1/1 -> q/1

== system s_b4a4x32kf_26/sys3/Delay12 ==
  d : Inport
  Register0 : xbsIndex_r4/Register  init=0  rst=off  en=off  dbl_ovrd=off  block_type=register
      settings: SourceProductName=The database /home/jmanley/.matlab/R2018a/slblocks_master.db is locked, or a table in the database is locked. (database is locked)  block_version=11.4
  Register1 : xbsIndex_r4/Register  init=0  rst=off  en=off  dbl_ovrd=off  block_type=register
      settings: SourceProductName=The database /home/jmanley/.matlab/R2018a/slblocks_master.db is locked, or a table in the database is locked. (database is locked)  block_version=11.4
  q : Outport
  wires:
  Register0/1 -> Register1/1
  d/1 -> Register0/1
  Register1/1 -> q/1

== system s_b4a4x32kf_26/sys3/Delay13 ==
  d : Inport
  Register0 : xbsIndex_r4/Register  init=0  rst=off  en=off  dbl_ovrd=off  block_type=register
      settings: SourceProductName=The database /home/jmanley/.matlab/R2018a/slblocks_master.db is locked, or a table in the database is locked. (database is locked)  block_version=11.4
  Register1 : xbsIndex_r4/Register  init=0  rst=off  en=off  dbl_ovrd=off  block_type=register
      settings: SourceProductName=The database /home/jmanley/.matlab/R2018a/slblocks_master.db is locked, or a table in the database is locked. (database is locked)  block_version=11.4
  q : Outport
  wires:
  Register0/1 -> Register1/1
  d/1 -> Register0/1
  Register1/1 -> q/1

== system s_b4a4x32kf_26/sys3/Delay14 ==
  d : Inport
  Register0 : xbsIndex_r4/Register  init=0  rst=off  en=off  dbl_ovrd=off  block_type=register
      settings: SourceProductName=The database /home/jmanley/.matlab/R2018a/slblocks_master.db is locked, or a table in the database is locked. (database is locked)  block_version=11.4
  Register1 : xbsIndex_r4/Register  init=0  rst=off  en=off  dbl_ovrd=off  block_type=register
      settings: SourceProductName=The database /home/jmanley/.matlab/R2018a/slblocks_master.db is locked, or a table in the database is locked. (database is locked)  block_version=11.4
  q : Outport
  wires:
  Register0/1 -> Register1/1
  d/1 -> Register0/1
  Register1/1 -> q/1

== system s_b4a4x32kf_26/sys3/Delay15 ==
  d : Inport
  Register0 : xbsIndex_r4/Register  init=0  rst=off  en=off  dbl_ovrd=off  block_type=register
      settings: SourceProductName=The database /home/jmanley/.matlab/R2018a/slblocks_master.db is locked, or a table in the database is locked. (database is locked)  block_version=11.4
  Register1 : xbsIndex_r4/Register  init=0  rst=off  en=off  dbl_ovrd=off  block_type=register
      settings: SourceProductName=The database /home/jmanley/.matlab/R2018a/slblocks_master.db is locked, or a table in the database is locked. (database is locked)  block_version=11.4
  q : Outport
  wires:
  Register0/1 -> Register1/1
  d/1 -> Register0/1
  Register1/1 -> q/1

== system s_b4a4x32kf_26/sys3/Delay16 ==
  d : Inport
  Register0 : xbsIndex_r4/Register  init=0  rst=off  en=off  dbl_ovrd=off  block_type=register
      settings: SourceProductName=The database /home/jmanley/.matlab/R2018a/slblocks_master.db is locked, or a table in the database is locked. (database is locked)  block_version=11.4
  Register1 : xbsIndex_r4/Register  init=0  rst=off  en=off  dbl_ovrd=off  block_type=register
      settings: SourceProductName=The database /home/jmanley/.matlab/R2018a/slblocks_master.db is locked, or a table in the database is locked. (database is locked)  block_version=11.4
  q : Outport
  wires:
  Register0/1 -> Register1/1
  d/1 -> Register0/1
  Register1/1 -> q/1

== system s_b4a4x32kf_26/sys3/Delay17 ==
  d : Inport
  Register0 : xbsIndex_r4/Register  init=0  rst=off  en=off  dbl_ovrd=off  block_type=register
      settings: SourceProductName=The database /home/jmanley/.matlab/R2018a/slblocks_master.db is locked, or a table in the database is locked. (database is locked)  block_version=11.4
  Register1 : xbsIndex_r4/Register  init=0  rst=off  en=off  dbl_ovrd=off  block_type=register
      settings: SourceProductName=The database /home/jmanley/.matlab/R2018a/slblocks_master.db is locked, or a table in the database is locked. (database is locked)  block_version=11.4
  q : Outport
  wires:
  Register0/1 -> Register1/1
  d/1 -> Register0/1
  Register1/1 -> q/1

== system s_b4a4x32kf_26/sys3/Delay18 ==
  d : Inport
  Register0 : xbsIndex_r4/Register  init=0  rst=off  en=off  dbl_ovrd=off  block_type=register
      settings: SourceProductName=The database /home/jmanley/.matlab/R2018a/slblocks_master.db is locked, or a table in the database is locked. (database is locked)  block_version=11.4
  Register1 : xbsIndex_r4/Register  init=0  rst=off  en=off  dbl_ovrd=off  block_type=register
      settings: SourceProductName=The database /home/jmanley/.matlab/R2018a/slblocks_master.db is locked, or a table in the database is locked. (database is locked)  block_version=11.4
  q : Outport
  wires:
  Register0/1 -> Register1/1
  d/1 -> Register0/1
  Register1/1 -> q/1

== system s_b4a4x32kf_26/sys3/Delay19 ==
  d : Inport
  Register0 : xbsIndex_r4/Register  init=0  rst=off  en=off  dbl_ovrd=off  block_type=register
      settings: SourceProductName=The database /home/jmanley/.matlab/R2018a/slblocks_master.db is locked, or a table in the database is locked. (database is locked)  block_version=11.4
  Register1 : xbsIndex_r4/Register  init=0  rst=off  en=off  dbl_ovrd=off  block_type=register
      settings: SourceProductName=The database /home/jmanley/.matlab/R2018a/slblocks_master.db is locked, or a table in the database is locked. (database is locked)  block_version=11.4
  q : Outport
  wires:
  Register0/1 -> Register1/1
  d/1 -> Register0/1
  Register1/1 -> q/1
